simulink model "Power_Plant"  (R2026b)
settings: Solver=VariableStepAuto
undefined symbols (not defined in the file or in its folder): Ts
settings Model: Creator=aomar  LastModifiedBy=aomar

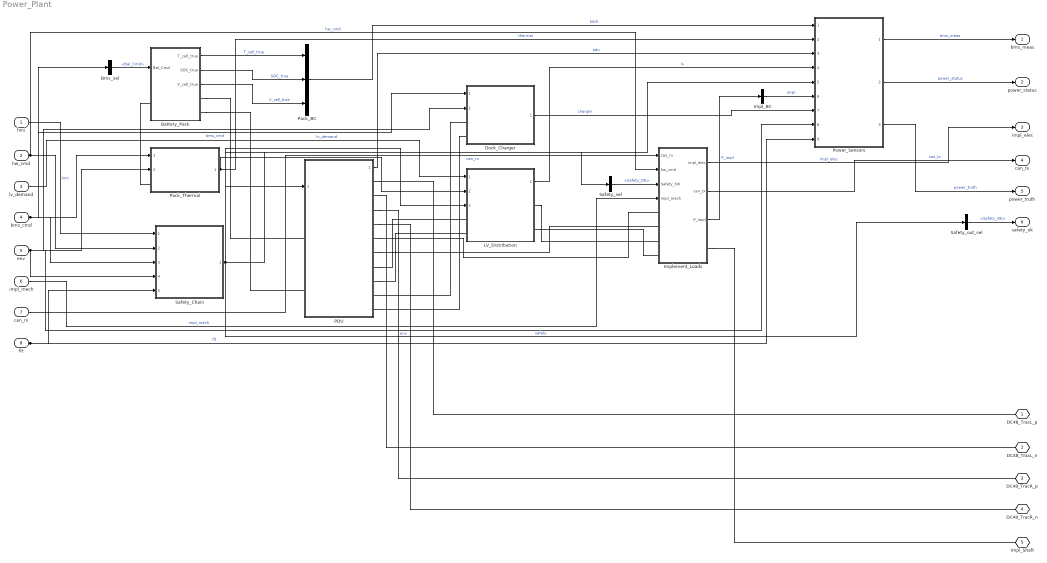
== system Power_Plant ==
  hmi : Inport  OutDataTypeStr=Bus: Bus_HmiInputs  SampleTime=Ts.base
  hw_cmd : Inport  Port=2  OutDataTypeStr=Bus: Bus_PowerHwCmd  SampleTime=Ts.base
  lv_demand : Inport  Port=3  OutDataTypeStr=Bus: Bus_LV_LoadDemand  SampleTime=Ts.ctrl
  bms_cmd : Inport  Port=4  OutDataTypeStr=Bus: Bus_BMS_Cmd  SampleTime=Ts.ctrl
  env : Inport  Port=5  OutDataTypeStr=Bus: Bus_EnvState  SampleTime=Ts.env
  impl_mech : Inport  Port=6  OutDataTypeStr=Bus: Bus_ImplMechState  SampleTime=Ts.ctrl
  can_rx : Inport  Port=7  OutDataTypeStr=Bus: Bus_Can1_McuSlow  SampleTime=Ts.can_slow
  flt : Inport  Port=8  OutDataTypeStr=Bus: Bus_FaultInject  SampleTime=Ts.base
  Battery_Pack : Subsystem  Variant=on
  Bms_sel : BusSelector  OutputSignals=Bal_Cmd
  Dock_Charger : Subsystem  ReferencedSubsystem=Dock_Charger
  Impl_BC : BusCreator  Inputs=1
  Implement_Loads : Subsystem  Variant=on
  LV_Distribution : Subsystem  ReferencedSubsystem=LV_Distribution
  PDU : Subsystem  ReferencedSubsystem=PDU
  Pack_BC : BusCreator  Inputs=3
  Pack_Thermal : Subsystem  ReferencedSubsystem=Pack_Thermal
  Power_Sensors : Subsystem  ReferencedSubsystem=Power_Sensors
  Safety_Chain : Subsystem  ReferencedSubsystem=Safety_Chain
  Safety_out_sel : BusSelector  OutputSignals=Safety_OK
  Safety_sel : BusSelector  OutputSignals=Safety_OK
  DC48_TracL_p : PMIOPort  Side=Right  ConnectionType=Connection: foundation.electrical.electrical
  DC48_TracL_n : PMIOPort  Port=2  Side=Right  ConnectionType=Connection: foundation.electrical.electrical
  DC48_TracR_p : PMIOPort  Port=3  Side=Right  ConnectionType=Connection: foundation.electrical.electrical
  DC48_TracR_n : PMIOPort  Port=4  Side=Right  ConnectionType=Connection: foundation.electrical.electrical
  Impl_Shaft : PMIOPort  Port=5  Side=Right  ConnectionType=Connection: foundation.mechanical.rotational.rotational
  bms_meas : Outport  OutDataTypeStr=Bus: Bus_BMS_Meas
  power_status : Outport  Port=2  OutDataTypeStr=Bus: Bus_PowerStatus
  impl_elec : Outport  Port=3  OutDataTypeStr=Bus: Bus_ImplElecState
  can_tx : Outport  Port=4  OutDataTypeStr=Bus: Bus_Can1_Impl
  power_truth : Outport  Port=5  OutDataTypeStr=Bus: Bus_PowerTruth
  safety_ok : Outport  Port=6  OutDataTypeStr=boolean
  wires:
  hmi/1 -> Safety_Chain/1  "hmi"
  hw_cmd/1 -> Safety_Chain/2, Implement_Loads/2(hw_cmd)  "hw_cmd"
  lv_demand/1 -> LV_Distribution/1  "lv_demand"
  bms_cmd/1 -> Bms_sel/1, Dock_Charger/1, Pack_Thermal/1, Safety_Chain/3  "bms_cmd"
  env/1 -> Dock_Charger/2, Power_Sensors/8, Pack_Thermal/2, Safety_Chain/4  "env"
  impl_mech/1 -> Implement_Loads/4(impl_mech)  "impl_mech"
  can_rx/1 -> Implement_Loads/1(can_rx)  "can_rx"
  flt/1 -> Power_Sensors/9, Safety_Chain/5  "flt"
  Bms_sel/1 -> Battery_Pack/1(Bal_Cmd)  "<Bal_Cmd>"
  Battery_Pack/1(T_cell_true) -> Pack_BC/1  "T_cell_true"
  Battery_Pack/2(SOC_true) -> Pack_BC/2  "SOC_true"
  Battery_Pack/3(V_cell_true) -> Pack_BC/3  "V_cell_true"
  Pack_Thermal/1 -> Power_Sensors/2, LV_Distribution/2  "thermal"
  Safety_Chain/1 -> Power_Sensors/5, Safety_sel/1, PDU/1, LV_Distribution/3, Safety_out_sel/1  "safety"
  Pack_BC/1 -> Power_Sensors/1  "pack"
  PDU/1 -> Power_Sensors/3  "pdu"
  Dock_Charger/1 -> Power_Sensors/7  "charger"
  LV_Distribution/1 -> Power_Sensors/4  "lv"
  Safety_sel/1 -> Implement_Loads/3(Safety_OK)  "<Safety_OK>"
  Implement_Loads/1(impl_elec) -> impl_elec/1  "impl_elec"
  Implement_Loads/2(can_tx) -> can_tx/1  "can_tx"
  Implement_Loads/3(P_impl) -> Impl_BC/1  "P_impl"
  Impl_BC/1 -> Power_Sensors/6  "impl"
  Power_Sensors/1 -> bms_meas/1  "bms_meas"
  Power_Sensors/2 -> power_status/1  "power_status"
  Power_Sensors/3 -> power_truth/1  "power_truth"
  Safety_out_sel/1 -> safety_ok/1  "<Safety_OK>"
  connections:
  Battery_Pack/LConn1 -- Pack_Thermal/LConn1
  Battery_Pack/RConn1 -- PDU/LConn1
  Battery_Pack/RConn2 -- PDU/LConn2
  PDU/RConn2 -- DC48_TracL_n/RConn1
  PDU/RConn1 -- DC48_TracL_p/RConn1
  PDU/RConn4 -- DC48_TracR_n/RConn1
  PDU/RConn3 -- DC48_TracR_p/RConn1
  Dock_Charger/LConn1 -- PDU/RConn9
  Dock_Charger/LConn2 -- PDU/RConn10
  Implement_Loads/RConn1 -- Impl_Shaft/RConn1
  PDU/RConn5 -- Implement_Loads/LConn1
  PDU/RConn6 -- Implement_Loads/LConn2
  LV_Distribution/RConn1 -- Implement_Loads/LConn3
  LV_Distribution/RConn2 -- Implement_Loads/LConn4
  PDU/RConn7 -- LV_Distribution/LConn1
  PDU/RConn8 -- LV_Distribution/LConn2

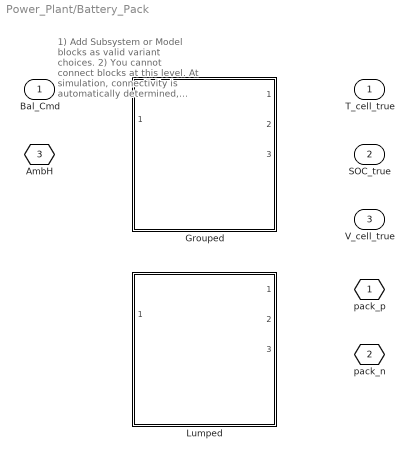
== system Power_Plant/Battery_Pack ==
  note: 1) Add Subsystem or Model blocks as valid variant choices.
      | 2) You cannot connect blocks at this level. At simulation, connectivity is automatically
      | determined, based on the active variant and port name matching.
  Bal_Cmd : Inport
  Grouped : Subsystem  VariantControl=VC_PACK == 1  ReferencedSubsystem=Pack_Grouped
  Lumped : Subsystem  VariantControl=VC_PACK == 2  ReferencedSubsystem=Pack_Lumped
  pack_p : PMIOPort  Side=Right  ConnectionType=Connection: foundation.electrical.electrical
  pack_n : PMIOPort  Port=2  Side=Right  ConnectionType=Connection: foundation.electrical.electrical
  AmbH : PMIOPort  Port=3  Side=Left  ConnectionType=Connection: foundation.thermal.thermal
  T_cell_true : Outport
  SOC_true : Outport  Port=2
  V_cell_true : Outport  Port=3

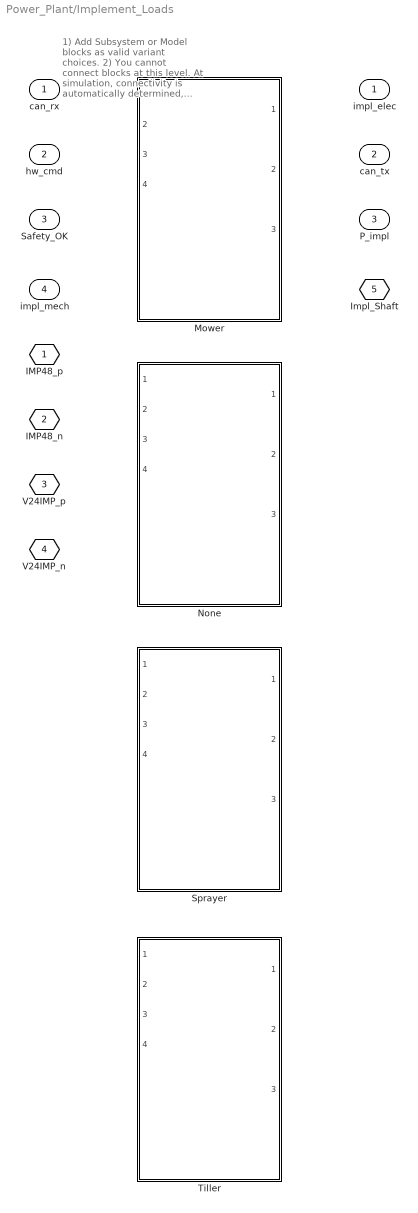
== system Power_Plant/Implement_Loads ==
  note: 1) Add Subsystem or Model blocks as valid variant choices.
      | 2) You cannot connect blocks at this level. At simulation, connectivity is automatically
      | determined, based on the active variant and port name matching.
  can_rx : Inport
  hw_cmd : Inport  Port=2
  Safety_OK : Inport  Port=3
  impl_mech : Inport  Port=4
  Mower : Subsystem  VariantControl=VC_IMPL == 1  ReferencedSubsystem=Impl_Mower
  None : Subsystem  VariantControl=VC_IMPL == 0  ReferencedSubsystem=Impl_None
  Sprayer : Subsystem  VariantControl=VC_IMPL == 3  ReferencedSubsystem=Impl_Sprayer
  Tiller : Subsystem  VariantControl=VC_IMPL == 2  ReferencedSubsystem=Impl_Tiller
  IMP48_p : PMIOPort  Side=Left  ConnectionType=Connection: foundation.electrical.electrical
  IMP48_n : PMIOPort  Port=2  Side=Left  ConnectionType=Connection: foundation.electrical.electrical
  V24IMP_p : PMIOPort  Port=3  Side=Left  ConnectionType=Connection: foundation.electrical.electrical
  V24IMP_n : PMIOPort  Port=4  Side=Left  ConnectionType=Connection: foundation.electrical.electrical
  Impl_Shaft : PMIOPort  Port=5  Side=Right  ConnectionType=Connection: foundation.mechanical.rotational.rotational
  impl_elec : Outport
  can_tx : Outport  Port=2
  P_impl : Outport  Port=3
